simulink model "gm_soc_dlmc_handshake_ddr"  (R2025b)
settings: Solver=FixedStepDiscrete  StartTime=0.0  StopTime=simTime  RelTol=1e-3
undefined symbols (not defined in the file or in its folder): sampleTimeDL
libraries: hdlsllib x3
settings Model: ModifiedByFormat=The MathWorks, Inc.  Creator=The MathWorks, Inc.  LastModifiedBy=The MathWorks, Inc.
settings SolverCC: PositivePriorityOrder=on
settings DataIOCC: SaveOutput=off  SaveTime=off
settings OptimizationCC: BlockReduction=off  ConditionallyExecuteInputs=off  DefaultParameterBehavior=Inlined  InheritOutputTypeSmallerThanSingle=on  EnhancedBackFolding=on  PassReuseOutputArgsAs=Individual arguments  ZeroExternalMemoryAtStartup=off  ZeroInternalMemoryAtStartup=off  MaxStackSize=64  OptimizeBlockOrder=speed  DifferentSizesBufferReuse=on  OptimizationCustomize=off  EfficientTunableParamExpr=on
settings DebuggingCC: ArtificialAlgebraicLoopMsg=error  InheritedTsInSrcMsg=none  SingleTaskRateTransMsg=error  ParameterTunabilityLossMsg=error  SubsystemReferenceDiagnosticForUnitTest=warning
settings HardwareCC: ProdBitPerPointer=32.0  ProdBitPerSizeT=32.0  ProdBitPerPtrDiffT=32.0  ProdLargestAtomicFloat=None  ProdIntDivRoundTo=Undefined  ProdEndianess=Unspecified  ProdWordSize=32.0  ProdHWDeviceType=ASIC/FPGA->ASIC/FPGA  TargetBitPerPointer=64.0  TargetBitPerSizeT=64.0  TargetBitPerPtrDiffT=64.0  TargetLongLongMode=on  TargetIntDivRoundTo=Zero  TargetEndianess=LittleEndian  TargetWordSize=64.0  TargetHWDeviceType=Custom Processor->MATLAB Host Computer  ProdEqTarget=off  HardwareBoardFeatureSet=SoCBlockset
settings ModelReferenceCC: EnableRefExpFcnMdlSchedulingChecks=on  ModelReferenceNumInstancesAllowed=Single
settings RTWCC: SystemTargetFile=ert.tlc  HardwareBoard=Xilinx Zynq UltraScale+ RFSoC ZCU111 Evaluation Kit  TLCOptions="-aInlineSetEventsForThisBaseRateFcn=TLC_FALSE -aSuppressMultiTaskScheduler=TLC_FALSE  -aRateBasedStepFcn=0"  TemplateMakefile=ert_default_tmf  Toolchain=Linaro AArch64 Linux v6.3.1  GPUComputeCapability=3.5  Description=Embedded Coder
settings CodeAppCC: ForceParamTrailComments=on  IgnoreCustomStorageClasses=off  OperatorAnnotations=on  SimulinkDataObjDesc=on  SFDataObjDesc=on  InsertBlockDesc=on
settings ERTTargetCC: CombineOutputUpdateFcns=off  SubcomponentCodeInterfacePackaging=Nonreusable function

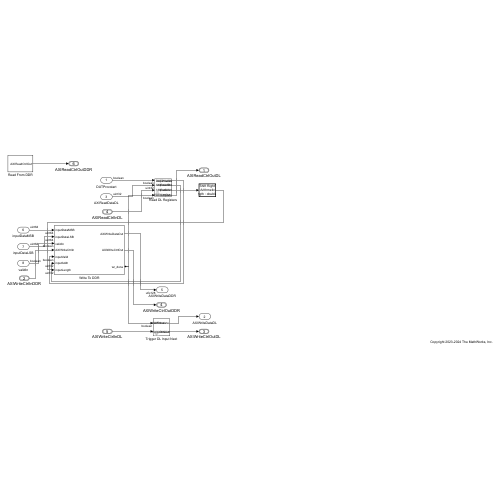
[thumbnail: Simulink's stored preview of the top-level diagram]
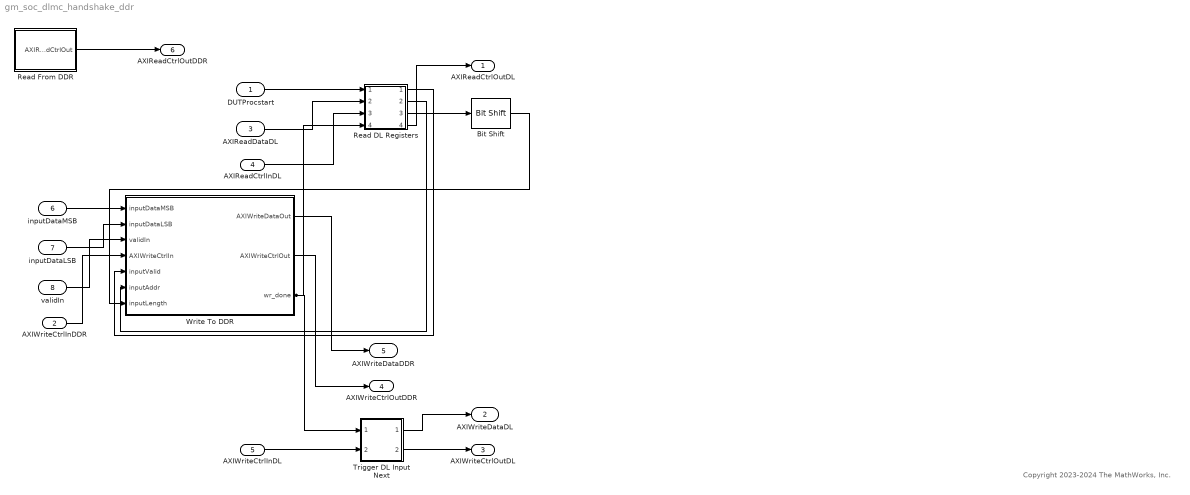
== system gm_soc_dlmc_handshake_ddr ==
  note: Copyright 2023-2024 The MathWorks, Inc.
  DUTProcstart : Inport  OutDataTypeStr=boolean  PortDimensions=1  SampleTime=3.90625e-09
  AXIWriteCtrlInDDR : Inport  Port=2  OutDataTypeStr=Bus: BusAXIWriteCtrlS2M  SampleTime=sampleTimeDL
  AXIReadDataDL : Inport  Port=3  OutDataTypeStr=uint32  PortDimensions=1  SampleTime=3.90625e-09
  AXIReadCtrlInDL : Inport  Port=4  OutDataTypeStr=Bus: BusAXIReadCtrlS2M  SampleTime=sampleTimeDL
  AXIWriteCtrlInDL : Inport  Port=5  OutDataTypeStr=Bus: BusAXIWriteCtrlS2M
  inputDataMSB : Inport  Port=6  OutDataTypeStr=fixdt(0, 64, 0)  PortDimensions=1  SampleTime=3.90625e-09
  inputDataLSB : Inport  Port=7  OutDataTypeStr=fixdt(0, 64, 0)  PortDimensions=1  SampleTime=3.90625e-09
  validIn : Inport  Port=8  OutDataTypeStr=boolean  PortDimensions=1  SampleTime=3.90625e-09
  Bit Shift : hdlsllib/Logic and Bit Operations/Bit Shift  mode=Shift Right Arithmetic  N=double(4)
  Read DL Registers : Subsystem  mask{ReadAddr=reshape(uint32([852;856;860]), [1  3])}
      mask prompts: ReadAddr "Read Address"
  Read From DDR : Subsystem
  Trigger DL Input Next : Subsystem  mask{DLDataIn=reshape(uint32([0;1;0]), [1  3]), DLAddrIn=reshape(uint32([848;848;848]), [1  3])}
      mask prompts: DLDataIn "Write Data"; DLAddrIn "Write Address"
  Write To DDR : Subsystem
  AXIReadCtrlOutDL : Outport  OutDataTypeStr=Bus: BusAXIReadCtrlM2S
  AXIWriteDataDL : Outport  Port=2  SampleTime=3.90625e-09
  AXIWriteCtrlOutDL : Outport  Port=3  OutDataTypeStr=Bus: BusAXIWriteCtrlM2S
  AXIWriteCtrlOutDDR : Outport  Port=4  OutDataTypeStr=Bus: BusAXIWriteCtrlM2S
  AXIWriteDataDDR : Outport  Port=5  OutDataTypeStr=fixdt(0, 4*bitWidth, 0)  SampleTime=3.90625e-09
  AXIReadCtrlOutDDR : Outport  Port=6  OutDataTypeStr=Bus: BusAXIReadCtrlM2S  VectorParamsAs1DForOutWhenUnconnected=off
  wires:
  Read From DDR/1(AXIReadCtrlOut) -> AXIReadCtrlOutDDR/1
  validIn/1 -> Write To DDR/3(validIn)
  inputDataMSB/1 -> Write To DDR/1(inputDataMSB)
  AXIWriteCtrlInDDR/1 -> Write To DDR/4(AXIWriteCtrlIn)
  AXIReadCtrlInDL/1 -> Read DL Registers/3(AXIReadCtrlIn)
  AXIWriteCtrlInDL/1 -> Trigger DL Input Next/2(AXIWriteCtrlIn)
  DUTProcstart/1 -> Read DL Registers/1(DUTProcStart)
  AXIReadDataDL/1 -> Read DL Registers/2(AXIReadData)
  inputDataLSB/1 -> Write To DDR/2(inputDataLSB)
  Write To DDR/1(AXIWriteDataOut) -> AXIWriteDataDDR/1
  Write To DDR/2(AXIWriteCtrlOut) -> AXIWriteCtrlOutDDR/1
  Write To DDR/3(wr_done) -> Trigger DL Input Next/1(wrDone), Read DL Registers/4(wrComplete)
  Read DL Registers/1(inputValid) -> Write To DDR/5(inputValid)
  Read DL Registers/2(inputAddr) -> Write To DDR/6(inputAddr)
  Read DL Registers/3(inputSize) -> Bit Shift/1
  Read DL Registers/4(AXIReadCtrlOut) -> AXIReadCtrlOutDL/1
  Trigger DL Input Next/1(AXIWritedata) -> AXIWriteDataDL/1
  Trigger DL Input Next/2(AXIWriteCtrlOut) -> AXIWriteCtrlOutDL/1
  Bit Shift/1 -> Write To DDR/7(inputLength)

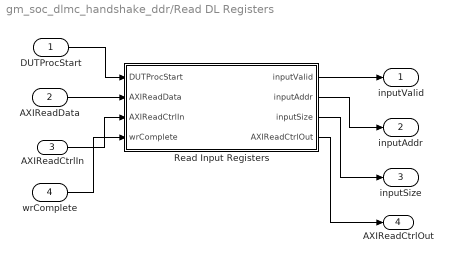
== system gm_soc_dlmc_handshake_ddr/Read DL Registers ==
  DUTProcStart : Inport  OutDataTypeStr=boolean  PortDimensions=1  SampleTime=3.90625e-09
  AXIReadData : Inport  Port=2  OutDataTypeStr=uint32  PortDimensions=1  SampleTime=3.90625e-09
  AXIReadCtrlIn : Inport  Port=3
  wrComplete : Inport  Port=4  OutDataTypeStr=boolean  PortDimensions=1  SampleTime=3.90625e-09
  Read Input Registers : Subsystem
  inputValid : Outport  SampleTime=3.90625e-09
  inputAddr : Outport  Port=2  SampleTime=3.90625e-09
  inputSize : Outport  Port=3  SampleTime=3.90625e-09
  AXIReadCtrlOut : Outport  Port=4
  wires:
  DUTProcStart/1 -> Read Input Registers/1(DUTProcStart)
  wrComplete/1 -> Read Input Registers/4(wrComplete)
  AXIReadCtrlIn/1 -> Read Input Registers/3(AXIReadCtrlIn)
  AXIReadData/1 -> Read Input Registers/2(AXIReadData)
  Read Input Registers/4(AXIReadCtrlOut) -> AXIReadCtrlOut/1
  Read Input Registers/3(inputSize) -> inputSize/1
  Read Input Registers/2(inputAddr) -> inputAddr/1
  Read Input Registers/1(inputValid) -> inputValid/1

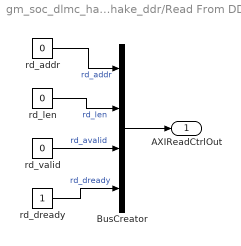
== system gm_soc_dlmc_handshake_ddr/Read From DDR ==
  BusCreator : BusCreator  Inputs=4
  rd_addr : Constant  Value=0  OutDataTypeStr=uint32  SampleTime=-1
  rd_dready : Constant  OutDataTypeStr=boolean  SampleTime=-1
  rd_len : Constant  Value=0  OutDataTypeStr=uint32  SampleTime=-1
  rd_valid : Constant  Value=0  OutDataTypeStr=boolean  SampleTime=-1
  AXIReadCtrlOut : Outport  VectorParamsAs1DForOutWhenUnconnected=off
  wires:
  rd_dready/1 -> BusCreator/4  "rd_dready"
  rd_valid/1 -> BusCreator/3  "rd_avalid"
  rd_len/1 -> BusCreator/2  "rd_len"
  rd_addr/1 -> BusCreator/1  "rd_addr"
  BusCreator/1 -> AXIReadCtrlOut/1

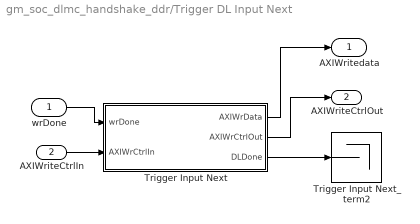
== system gm_soc_dlmc_handshake_ddr/Trigger DL Input Next ==
  wrDone : Inport  OutDataTypeStr=boolean  PortDimensions=1  SampleTime=3.90625e-09
  AXIWriteCtrlIn : Inport  Port=2
  Trigger Input Next : Subsystem
  Trigger Input Next_term2 : Terminator
  AXIWritedata : Outport  SampleTime=3.90625e-09  VectorParamsAs1DForOutWhenUnconnected=off
  AXIWriteCtrlOut : Outport  Port=2  VectorParamsAs1DForOutWhenUnconnected=off
  wires:
  AXIWriteCtrlIn/1 -> Trigger Input Next/2(AXIWrCtrlIn)
  wrDone/1 -> Trigger Input Next/1(wrDone)
  Trigger Input Next/1(AXIWrData) -> AXIWritedata/1
  Trigger Input Next/3(DLDone) -> Trigger Input Next_term2/1
  Trigger Input Next/2(AXIWrCtrlOut) -> AXIWriteCtrlOut/1

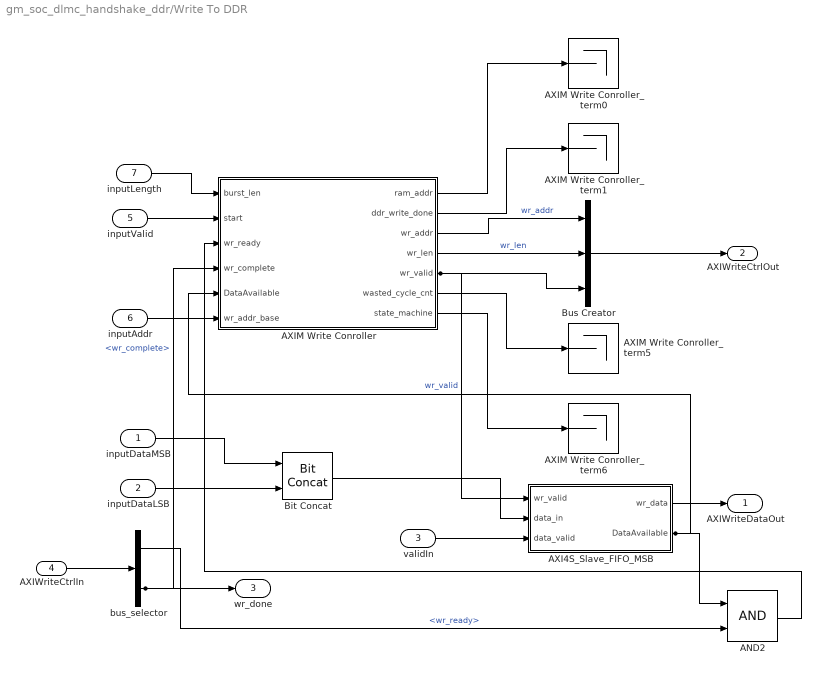
== system gm_soc_dlmc_handshake_ddr/Write To DDR ==
  inputDataMSB : Inport  OutDataTypeStr=fixdt(0, 64, 0)  PortDimensions=1  SampleTime=3.90625e-09
  inputDataLSB : Inport  Port=2  OutDataTypeStr=fixdt(0, 64, 0)  PortDimensions=1  SampleTime=3.90625e-09
  validIn : Inport  Port=3  OutDataTypeStr=boolean  PortDimensions=1  SampleTime=3.90625e-09
  AXIWriteCtrlIn : Inport  Port=4
  inputValid : Inport  Port=5  OutDataTypeStr=boolean  PortDimensions=1  SampleTime=3.90625e-09
  inputAddr : Inport  Port=6  OutDataTypeStr=uint32  PortDimensions=1  SampleTime=3.90625e-09
  inputLength : Inport  Port=7  OutDataTypeStr=uint32  PortDimensions=1  SampleTime=3.90625e-09
  AND2 : Logic  AllPortsSameDT=off  OutDataTypeStr=boolean  SampleTime=3.90625e-09
  AXI4S_Slave_FIFO_MSB : Subsystem
  AXIM Write Conroller : Subsystem
  AXIM Write Conroller_term{0..1,5..6} (4 alike) : Terminator
  Bit Concat : hdlsllib/Logic and Bit Operations/Bit Concat  numInputs=2
  Bus Creator : BusCreator  Inputs=3
  bus_selector : BusSelector  OutputSignals=wr_ready,wr_complete
  AXIWriteDataOut : Outport  SampleTime=3.90625e-09
  AXIWriteCtrlOut : Outport  Port=2
  wr_done : Outport  Port=3  SampleTime=3.90625e-09
  wires:
  inputValid/1 -> AXIM Write Conroller/2(start)
  AXIWriteCtrlIn/1 -> bus_selector/1
  inputAddr/1 -> AXIM Write Conroller/6(wr_addr_base)
  inputLength/1 -> AXIM Write Conroller/1(burst_len)
  inputDataLSB/1 -> Bit Concat/2
  inputDataMSB/1 -> Bit Concat/1
  bus_selector/2 -> wr_done/1, AXIM Write Conroller/4(wr_complete)  "<wr_complete>"
  bus_selector/1 -> AND2/2  "<wr_ready>"
  AXIM Write Conroller/5(wr_valid) -> Bus Creator/3, AXI4S_Slave_FIFO_MSB/1(wr_valid)  "wr_valid"
  AXIM Write Conroller/1(ram_addr) -> AXIM Write Conroller_term0/1
  AXIM Write Conroller/2(ddr_write_done) -> AXIM Write Conroller_term1/1
  AXIM Write Conroller/3(wr_addr) -> Bus Creator/1  "wr_addr"
  AXIM Write Conroller/4(wr_len) -> Bus Creator/2  "wr_len"
  AXIM Write Conroller/6(wasted_cycle_cnt) -> AXIM Write Conroller_term5/1
  AXIM Write Conroller/7(state_machine) -> AXIM Write Conroller_term6/1
  Bit Concat/1 -> AXI4S_Slave_FIFO_MSB/2(data_in)
  validIn/1 -> AXI4S_Slave_FIFO_MSB/3(data_valid)
  Bus Creator/1 -> AXIWriteCtrlOut/1
  AXI4S_Slave_FIFO_MSB/1(wr_data) -> AXIWriteDataOut/1
  AXI4S_Slave_FIFO_MSB/2(DataAvailable) -> AXIM Write Conroller/5(DataAvailable), AND2/1
  AND2/1 -> AXIM Write Conroller/3(wr_ready)

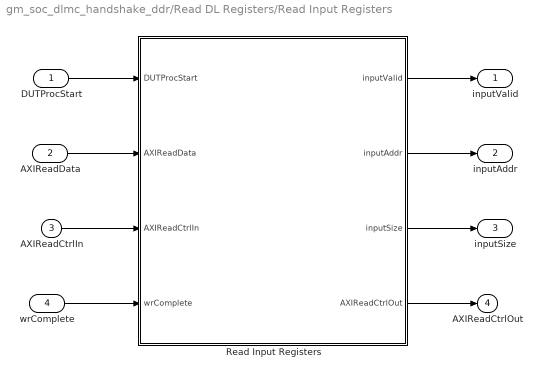
== system gm_soc_dlmc_handshake_ddr/Read DL Registers/Read Input Registers ==
  DUTProcStart : Inport  OutDataTypeStr=boolean  PortDimensions=1  SampleTime=3.90625e-09
  AXIReadData : Inport  Port=2  OutDataTypeStr=uint32  PortDimensions=1  SampleTime=3.90625e-09
  AXIReadCtrlIn : Inport  Port=3
  wrComplete : Inport  Port=4  OutDataTypeStr=boolean  PortDimensions=1  SampleTime=3.90625e-09
  Read Input Registers : MATLAB Function  TreatAsAtomicUnit=on
  inputValid : Outport  SampleTime=3.90625e-09
  inputAddr : Outport  Port=2  SampleTime=3.90625e-09
  inputSize : Outport  Port=3  SampleTime=3.90625e-09
  AXIReadCtrlOut : Outport  Port=4  VectorParamsAs1DForOutWhenUnconnected=off
  wires:
  wrComplete/1 -> Read Input Registers/4(wrComplete)
  AXIReadCtrlIn/1 -> Read Input Registers/3(AXIReadCtrlIn)
  AXIReadData/1 -> Read Input Registers/2(AXIReadData)
  DUTProcStart/1 -> Read Input Registers/1(DUTProcStart)
  Read Input Registers/4(AXIReadCtrlOut) -> AXIReadCtrlOut/1
  Read Input Registers/3(inputSize) -> inputSize/1
  Read Input Registers/2(inputAddr) -> inputAddr/1
  Read Input Registers/1(inputValid) -> inputValid/1

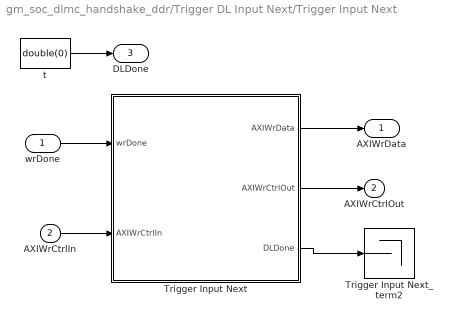
== system gm_soc_dlmc_handshake_ddr/Trigger DL Input Next/Trigger Input Next ==
  wrDone : Inport  OutDataTypeStr=boolean  PortDimensions=1  SampleTime=3.90625e-09
  AXIWrCtrlIn : Inport  Port=2
  Trigger Input Next : MATLAB Function  TreatAsAtomicUnit=on
  Trigger Input Next_term2 : Terminator
  t : Constant  Value=double(0)  OutDataTypeStr=boolean  SampleTime=3.90625e-09
  AXIWrData : Outport  SampleTime=3.90625e-09  VectorParamsAs1DForOutWhenUnconnected=off
  AXIWrCtrlOut : Outport  Port=2  VectorParamsAs1DForOutWhenUnconnected=off
  DLDone : Outport  Port=3  SampleTime=3.90625e-09  VectorParamsAs1DForOutWhenUnconnected=off
  wires:
  AXIWrCtrlIn/1 -> Trigger Input Next/2(AXIWrCtrlIn)
  wrDone/1 -> Trigger Input Next/1(wrDone)
  t/1 -> DLDone/1
  Trigger Input Next/3(DLDone) -> Trigger Input Next_term2/1
  Trigger Input Next/2(AXIWrCtrlOut) -> AXIWrCtrlOut/1
  Trigger Input Next/1(AXIWrData) -> AXIWrData/1

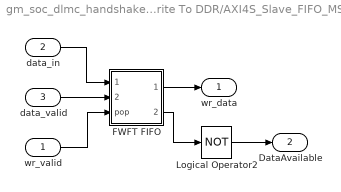
== system gm_soc_dlmc_handshake_ddr/Write To DDR/AXI4S_Slave_FIFO_MSB ==
  wr_valid : Inport  OutDataTypeStr=boolean  PortDimensions=1  SampleTime=3.90625e-09
  data_in : Inport  Port=2  OutDataTypeStr=fixdt(0, 128, 0)  PortDimensions=1  SampleTime=3.90625e-09
  data_valid : Inport  Port=3  OutDataTypeStr=boolean  PortDimensions=1  SampleTime=3.90625e-09
  FWFT FIFO : Subsystem  mask{FIFO_DEPTH=double(3072), AFULL_THRESH=double(200)}
      mask prompts: FIFO_DEPTH "FIFO Depth:"; AFULL_THRESH "Almost Full Threshold:"
  Logical Operator2 : Logic  Operator=NOT  IconShape=distinctive  AllPortsSameDT=off  OutDataTypeStr=boolean
  wr_data : Outport  SampleTime=3.90625e-09
  DataAvailable : Outport  Port=2  SampleTime=3.90625e-09
  wires:
  wr_valid/1 -> FWFT FIFO/3(pop)
  data_in/1 -> FWFT FIFO/1(data_i)
  data_valid/1 -> FWFT FIFO/2(push)
  FWFT FIFO/2(empty_o) -> Logical Operator2/1
  FWFT FIFO/1(data_o) -> wr_data/1
  Logical Operator2/1 -> DataAvailable/1

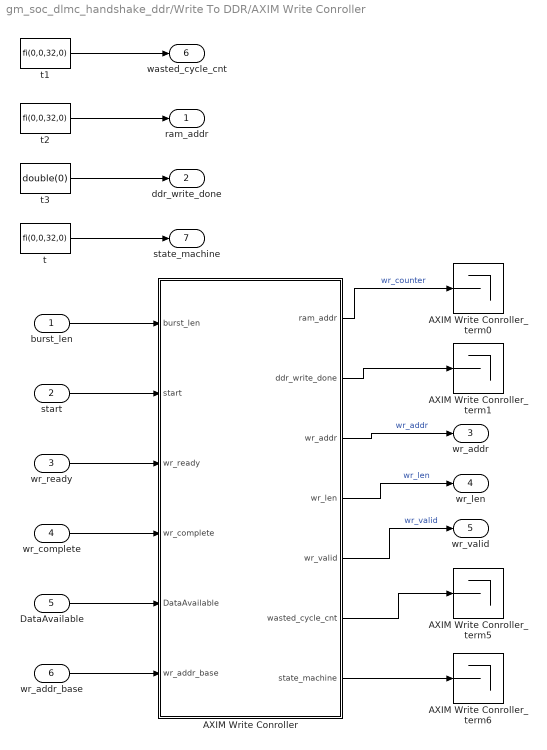
== system gm_soc_dlmc_handshake_ddr/Write To DDR/AXIM Write Conroller ==
  burst_len : Inport  OutDataTypeStr=uint32  PortDimensions=1  SampleTime=3.90625e-09
  start : Inport  Port=2  OutDataTypeStr=boolean  PortDimensions=1  SampleTime=3.90625e-09
  wr_ready : Inport  Port=3  OutDataTypeStr=boolean  PortDimensions=1  SampleTime=3.90625e-09
  wr_complete : Inport  Port=4  OutDataTypeStr=boolean  PortDimensions=1  SampleTime=3.90625e-09
  DataAvailable : Inport  Port=5  OutDataTypeStr=boolean  PortDimensions=1  SampleTime=3.90625e-09
  wr_addr_base : Inport  Port=6  OutDataTypeStr=uint32  PortDimensions=1  SampleTime=3.90625e-09
  AXIM Write Conroller : MATLAB Function  TreatAsAtomicUnit=on
  AXIM Write Conroller_term{0..1,5..6} (4 alike) : Terminator
  t : Constant  Value=fi(0,0,32,0)  OutDataTypeStr=uint32  SampleTime=3.90625e-09
  t1 : Constant  Value=fi(0,0,32,0)  OutDataTypeStr=uint32  SampleTime=3.90625e-09
  t2 : Constant  Value=fi(0,0,32,0)  OutDataTypeStr=uint32  SampleTime=3.90625e-09
  t3 : Constant  Value=double(0)  OutDataTypeStr=boolean  SampleTime=3.90625e-09
  ram_addr : Outport  SampleTime=3.90625e-09  VectorParamsAs1DForOutWhenUnconnected=off
  ddr_write_done : Outport  Port=2  SampleTime=3.90625e-09  VectorParamsAs1DForOutWhenUnconnected=off
  wr_addr : Outport  Port=3  SampleTime=3.90625e-09  VectorParamsAs1DForOutWhenUnconnected=off
  wr_len : Outport  Port=4  SampleTime=3.90625e-09  VectorParamsAs1DForOutWhenUnconnected=off
  wr_valid : Outport  Port=5  SampleTime=3.90625e-09  VectorParamsAs1DForOutWhenUnconnected=off
  wasted_cycle_cnt : Outport  Port=6  SampleTime=3.90625e-09  VectorParamsAs1DForOutWhenUnconnected=off
  state_machine : Outport  Port=7  SampleTime=3.90625e-09  VectorParamsAs1DForOutWhenUnconnected=off
  wires:
  t2/1 -> ram_addr/1
  t/1 -> state_machine/1
  t1/1 -> wasted_cycle_cnt/1
  t3/1 -> ddr_write_done/1
  burst_len/1 -> AXIM Write Conroller/1(burst_len)
  wr_complete/1 -> AXIM Write Conroller/4(wr_complete)
  wr_ready/1 -> AXIM Write Conroller/3(wr_ready)
  wr_addr_base/1 -> AXIM Write Conroller/6(wr_addr_base)
  start/1 -> AXIM Write Conroller/2(start)
  DataAvailable/1 -> AXIM Write Conroller/5(DataAvailable)
  AXIM Write Conroller/1(ram_addr) -> AXIM Write Conroller_term0/1  "wr_counter"
  AXIM Write Conroller/2(ddr_write_done) -> AXIM Write Conroller_term1/1
  AXIM Write Conroller/3(wr_addr) -> wr_addr/1  "wr_addr"
  AXIM Write Conroller/4(wr_len) -> wr_len/1  "wr_len"
  AXIM Write Conroller/5(wr_valid) -> wr_valid/1  "wr_valid"
  AXIM Write Conroller/6(wasted_cycle_cnt) -> AXIM Write Conroller_term5/1
  AXIM Write Conroller/7(state_machine) -> AXIM Write Conroller_term6/1

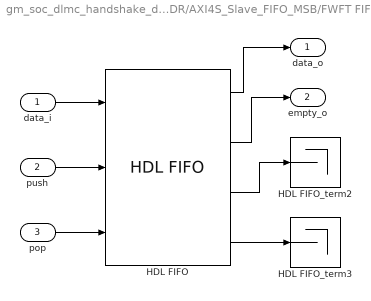
== system gm_soc_dlmc_handshake_ddr/Write To DDR/AXI4S_Slave_FIFO_MSB/FWFT FIFO ==
  data_i : Inport  OutDataTypeStr=fixdt(0, 128, 0)  PortDimensions=1  SampleTime=3.90625e-09
  push : Inport  Port=2  OutDataTypeStr=boolean  PortDimensions=1  SampleTime=3.90625e-09
  pop : Inport  Port=3  OutDataTypeStr=boolean  PortDimensions=1  SampleTime=3.90625e-09
  HDL FIFO : hdlsllib/HDL RAMs/HDL FIFO  fifo_size=FIFO_DEPTH  mode=FWFT  ratio=1  push_msg=Ignore  pop_msg=Ignore  show_empty=on  show_full=on  show_num=on  LabelModeActiveChoice_Mode=FWFT  rst_port=off
  HDL FIFO_term2 : Terminator
  HDL FIFO_term3 : Terminator
  data_o : Outport  SampleTime=3.90625e-09
  empty_o : Outport  Port=2  SampleTime=3.90625e-09
  wires:
  push/1 -> HDL FIFO/2
  data_i/1 -> HDL FIFO/1
  pop/1 -> HDL FIFO/3
  HDL FIFO/2 -> empty_o/1
  HDL FIFO/1 -> data_o/1
  HDL FIFO/4 -> HDL FIFO_term3/1
  HDL FIFO/3 -> HDL FIFO_term2/1

== matlab function gm_soc_dlmc_handshake_ddr/Write To DDR/AXIM Write Conroller/AXIM Write Conroller ==
  data: ram_addr output; ddr_write_done output; burst_len input; start input boolean; wr_ready input; wr_complete input; DataAvailable input; wr_addr output; wr_len output; wr_valid output; wasted_cycle_cnt output; state_machine output; wr_addr_base input
function [ram_addr, ddr_write_done, wr_addr, wr_len, wr_valid, wasted_cycle_cnt,state_machine] = ...
    hdlcoder_external_memory_write_ctrl(burst_len, start, wr_ready, wr_complete, DataAvailable,...
                                        wr_addr_base)

% create persistent variables (registers)
persistent wstate burst_stop burst_count burst_wr_addr wasted_cycle_count

if(isempty(wstate))
    wstate      = fi(0, 0, 4, 0);
    burst_stop  = uint32(0);
    burst_count = uint32(0);
    burst_wr_addr = uint32(0);
    wasted_cycle_count = uint32(0);    
end

wasted_cycle_cnt = cast(0,'like',wasted_cycle_count);
state_machine = uint32(0);

% state machine encoding
IDLE              = fi(0, 0, 4, 0);
WRITE_BURST_START = fi(1, 0, 4, 0);
DATA_COUNT        = fi(2, 0, 4, 0);
ACK_WAIT          = fi(3, 0, 4, 0);

% state machine logic
switch (wstate)
    case IDLE
        % output to AXI4 Master
        wr_addr  = uint32(0);
        wr_len   = uint32(0);
        wr_valid = false;
        
        % output to DUT logic
        ram_addr = uint32(0);
        ddr_write_done = true;
        
        % state variables
        burst_wr_addr = uint32(wr_addr_base);
        burst_stop  = uint32(burst_len);
        burst_count = uint32(0);
        
        if start
            wstate(:) = WRITE_BURST_START;
        else
            wstate(:) = IDLE;
        end
        
        
    case WRITE_BURST_START
        % output to AXI4 Master
        wr_addr  = uint32(burst_wr_addr);
        wr_len   = uint32(burst_stop);
        wr_valid = false;
        
        % output to DUT logic
        ram_addr = uint32(burst_count);
        ddr_write_done = false;
    
        
        if wr_ready
            wstate(:) = DATA_COUNT;
        else
            wstate(:) = WRITE_BURST_START;
            wasted_cycle_count = uint32(wasted_cycle_count+1);
        end
        
        
    case DATA_COUNT
        % output to AXI4 Master
        wr_addr  = uint32(burst_wr_addr);
        wr_len   = uint32(burst_stop);
        wr_valid = true && DataAvailable;
        
        % state variables
        if DataAvailable
            burst_count = uint32(burst_count + 1);
        end
        
        % output to DUT logic
        ram_addr = uint32(burst_count);
        ddr_write_done = false;
        
        if ( burst_count == burst_stop )
            wstate(:) = ACK_WAIT;
        else
            if ( wr_ready )
                wstate(:) = DATA_COUNT;
            else
                wstate(:) = WRITE_BURST_START;
            end
        end
        
        
    case ACK_WAIT
        % output to AXI4 Master
        wr_addr  = uint32(0);
        wr_len   = uint32(0);
        wr_valid = false;
        
        % output to DUT logic
        ram_addr = uint32(0);
        ddr_write_done = false;
        
        if wr_complete
            wstate(:) = IDLE;
        else
            wstate(:) = ACK_WAIT;
        end
        
    otherwise
        % output to AXI4 Master
        wr_addr = uint32(0);
        wr_len = uint32(0);
        wr_valid = false;
        
        % output to DUT logic
        ram_addr = uint32(0);
        ddr_write_done = false;
        
        wstate(:) = IDLE;
        
end
    
% For AXI4 MM Diagonstics
wasted_cycle_cnt(:) = wasted_cycle_count;
state_machine(:) = wstate;
end

% LocalWords:  AXI

== matlab function gm_soc_dlmc_handshake_ddr/Read DL Registers/Read Input Registers/Read Input Registers ==
  data: inputValid output; inputAddr output; inputSize output; DUTProcStart input; AXIReadData input; AXIReadCtrlOut output Bus: BusAXIReadCtrlM2S; AXIReadCtrlIn input Bus: BusAXIReadCtrlS2M; ReadAddr parameter; wrComplete input
function [inputValid, inputAddr, inputSize, AXIReadCtrlOut] = ReadInputRegisters(DUTProcStart, AXIReadData, AXIReadCtrlIn, ReadAddr,wrComplete)

% Declare states of the FSM
IDLE = fi(0,0,4,0);
READ_AREADY_VALID = fi(1,0,4,0);
RD_VALID_WAIT = fi(2,0,4,0);
WAIT_WR_COMPLETE = fi(3,0,4,0);


persistent state cnt rdaddr rdavalid b_inputValid b_inputSize b_inputAddr all_valid
if isempty(state)
    state = IDLE;
    rdavalid = false;
    rdaddr = uint32(0);
    b_inputValid = uint32(0);
    b_inputSize = uint32(0);
    b_inputAddr = uint32(0);
    cnt = fi(1,0,8,0);
    all_valid = false;
end

AXIReadCtrlOut = struct('rd_addr', rdaddr, 'rd_len', uint32(1), 'rd_avalid', rdavalid, 'rd_dready', true );
inputValid = false;

% Assert inputValid only when all_valid is true
if(all_valid)
    inputValid = (b_inputValid ~= 0);
end

inputAddr = b_inputAddr;
inputSize = b_inputSize;


switch state
    % IDLE state resets the parameters of FSM
    case IDLE
        rdavalid = false;
        rdaddr = uint32(0);
        cnt = fi(1,0,8,0);
        all_valid = false;

        % Switch to the next state when DUTProcStart is asserted
        if DUTProcStart
            cnt(:) = 1;
            rdaddr = ReadAddr(cnt);
            if AXIReadCtrlIn.rd_aready
                rdavalid = true;
                state = RD_VALID_WAIT;
            else
                state = READ_AREADY_VALID;
            end
        end

    case READ_AREADY_VALID
        if AXIReadCtrlIn.rd_aready
            rdaddr = ReadAddr(cnt);
            rdavalid = true;
            state = RD_VALID_WAIT;
        end


    % RD_VALID_WAIT state reads the Input Registers of DLIP
    case RD_VALID_WAIT
        if AXIReadCtrlIn.rd_dvalid
            % Read InputValid Register from DLIP
            if(cnt == 1)
                all_valid = false;
                b_inputValid = AXIReadData;
                if(b_inputValid == 1)
                    cnt(:) = cnt + 1;
                    rdaddr = ReadAddr(cnt);
                    if AXIReadCtrlIn.rd_aready
                        rdavalid = true;
                        state = RD_VALID_WAIT;
                    else
                        state = READ_AREADY_VALID;
                    end
                else
                    state = READ_AREADY_VALID;
                end

            % Read InputAddr Register from DLIP
            elseif(cnt==2)
                all_valid = false;
                b_inputAddr = uint32(AXIReadData);
                cnt(:) = cnt + 1;
                rdaddr = ReadAddr(cnt);
                if AXIReadCtrlIn.rd_aready
                    rdavalid = true;
                    state = RD_VALID_WAIT;
                else
                    state = READ_AREADY_VALID;
                    cnt = fi(1,0,8,0);
                end

                % Read InputSize Register from DLIP
            elseif(cnt==3)
                all_valid = true;
                b_inputSize = uint32(AXIReadData);
                state = WAIT_WR_COMPLETE;
                cnt(:) = fi(1,0,8,0);
            else
                state = READ_AREADY_VALID;
                cnt(:) = fi(1,0,8,0);
            end
        else
            rdavalid = false;
        end



    % Wait for the current frame to be written before reading the registers
    % of next frame
    case WAIT_WR_COMPLETE
        rdavalid = false;
        all_valid= false;
        if(wrComplete==1)
            state = IDLE;
        end


    otherwise
        state = IDLE;
        rdavalid = false;
        rdaddr = uint32(0);
        b_inputValid = uint32(0);
        b_inputSize = uint32(0);
        b_inputAddr = uint32(0);
        cnt = fi(1,0,8,0);
        all_valid = false;


end
end

== matlab function gm_soc_dlmc_handshake_ddr/Trigger DL Input Next/Trigger Input Next/Trigger Input Next ==
  data: AXIWrData output; AXIWrCtrlOut output Bus: BusAXIWriteCtrlM2S; wrDone input; AXIWrCtrlIn input Bus: BusAXIWriteCtrlS2M; DLDone output; DLDataIn parameter; DLAddrIn parameter
function [AXIWrData, AXIWrCtrlOut, DLDone] = TriggerInputNext(wrDone, AXIWrCtrlIn, DLDataIn, DLAddrIn)

IDLE = fi(0,0,4,0);
WR_READY_WAIT = fi(1,0,4,0);
WR_COMPLETE_WAIT = fi(3,0,4,0);

persistent state cnt numdata wrdata wraddr wrvalid wrdone

if isempty(state)
    state = IDLE;
    numdata = fi(numel(DLDataIn),0,8,0);
    cnt = fi(1,0,8,0);
    wrdata = uint32(0);
    wraddr = uint32(0);
    wrvalid = false;
    wrdone = false;
end

AXIWrData = wrdata;
AXIWrCtrlOut = struct('wr_addr', wraddr, 'wr_len', uint32(1), 'wr_valid', wrvalid);
DLDone = wrdone;
wrvalid = false;
wrdone = false;

switch state
    case IDLE
        if wrDone
            cnt(:) = 1;
            wrdata = DLDataIn(cnt);
            wraddr = DLAddrIn(cnt);
            if AXIWrCtrlIn.wr_ready
                wrvalid = true;
                state = WR_COMPLETE_WAIT;
            else
                state = WR_READY_WAIT;
            end
        end
    case WR_READY_WAIT
        if AXIWrCtrlIn.wr_ready
            wrvalid = true;
            state = WR_COMPLETE_WAIT;
        end
    case WR_COMPLETE_WAIT
        if AXIWrCtrlIn.wr_complete
            if cnt == numdata
                state = IDLE;
                wrdone = true;
            else
                cnt(:) = cnt + 1;
                wrdata = DLDataIn(cnt);
                wraddr = DLAddrIn(cnt);
                if AXIWrCtrlIn.wr_ready
                    wrvalid = true;
                    state = WR_COMPLETE_WAIT;
                else
                    state = WR_READY_WAIT;
                end
            end
        end
    otherwise
end
